simulink model "EV6_LUT_FourWheel_EV6Battery77p4kWh_PowerCorrected"  (R2024a)
settings: Solver=ode4  StartTime=0  StopTime=60  FixedStep=0.001  RelTol=1e-3
PreLoadFcn:
  | VSS_BICYCLE=Simulink.Variant('Dual=0');
  | VSS_DUAL=Simulink.Variant('Dual=1');
  | Dual=1;
  | load('DriveCycle2.mat')
PostLoadFcn:
  | if any(exist('dsrtsu_mdlpostloadfcn', 'file') ~= 0), dsrtsu_mdlpostloadfcn('Execute', bdroot); end
InitFcn:
  | , if any(exist('rtifpga_mdlclblib', 'file') ~= 0), rtifpga_mdlclblib('Init', bdroot); end,
  | , if any(exist('dsmpb_private', 'file') ~= 0), dsmpb_private('dsmpb_mdlclblib', 'Init', bdroot); end,
  | load('DriveCycle2.mat')
model workspace (MAT data in the model file):
  DiffRatio = 10.65
  EV6_2023_BattBranchCapacity_Ah = 55.5236728838
  EV6_2023_BattEnergy_kWh = 77.4
  EV6_2023_BattNominalVoltage_V = 697
  EV6_2023_BattNumCellsParallel = 2
  EV6_2023_BattNumCellsSeries = 192
  EV6_2023_BattOpenVoltCapBpts = [0 0.1 0.2 0.3 0.4 0.5 0.6 0.7 0.8 0.9 1]
  EV6_2023_BattOpenVoltTbl = [2.96762142548 3.40364281191 3.47417488548 3.54470541822 3.61523441014 3.68576186124 3.75628777151 3.82681214095 3.94527005036 4.07101207308 4.2120755254]
  EV6_2023_BattPackCapacity_Ah = 111.047345768
  EV6_2023_BattResistSocBpts = [0 0.2 0.4 0.6 0.8 1]
  EV6_2023_BattResistTbl = [0.0163620057716 0.0118174152018 0.00807187352333 0.00375663957972 0.00266904525531 0.00103635901355 0.0019014404175 0.0172368903217 0.0121226074867 0.00758541551769 0.00474065349228 0.00337561163613 ... (42 elements, 7x6)]
  EV6_2023_BattResistTempBpts = [243.1 253.1 263.1 273.1 283.1 298.1 313.1]
  EV6_2023_InitialPackOCV_V = 726.471714233
  EV6_2023_InitialSOC = 0.638878863672
  EV6_BattCellCapacity_Ah = 60.3
  EV6_BattInitialSOC = 0.638878863672
  EV6_BattOCV_Cell_V = [2.96762142548 3.40364281191 3.47417488548 3.54470541822 3.61523441014 3.68576186124 3.75628777151 3.82681214095 3.94527005036 4.07101207308 4.2120755254]
  EV6_BattOCV_SOC = [0 0.1 0.2 0.3 0.4 0.5 0.6 0.7 0.8 0.9 1]
  EV6_BattPackCapacity_Ah = 120.6
  EV6_BattParallelCells = 2
  EV6_BattResistanceSOC = [0 0.2 0.4 0.6 0.8 1]
  EV6_BattResistanceTable_Ohm = [0.0163620057716 0.0118174152018 0.00807187352333 0.00375663957972 0.00266904525531 0.00103635901355 0.0019014404175 0.0172368903217 0.0121226074867 0.00758541551769 0.00474065349228 0.00337561163613 ... (42 elements, 7x6)]
  EV6_BattResistanceTemp_K = [243.1 253.1 263.1 273.1 283.1 298.1 313.1]
  EV6_BattSeriesCells = 192
  EV6_FinalDriveRatio = 10.65
  EV6_TargetPackResistance_Ohm = 0.132763804608
  Gas = 0.383333333333
undefined symbols (not defined in the file): accel_bp_mps2, AccelCmd, ActTqLF_Nm_, ActTqLR_Nm_, ActTqRF_Nm_, ActTqRR_Nm_, BattChargeLimitMaxPwr, BattChargeLimitSocBpts, BattChargeLimitTbl, BattDischargeLimitSocBpts, BattDischargeLimitTbl, BattDischargeMaxPwr, BrakeMaxPrs, BrakeMaxTrq, ChassisDistCg2FrontAxle, ChassisDistCg2RearAxle, ChassisVehMass, CltchCmd, CoastDown, DecelCmd, DiscIntNeverNeededParam, EnvGravCnst, EnvPrs, EnvTemp, EV6_RegenTorqueGain, EV6_TractionTorqueGain, front_share_regen_3d, front_share_traction_3d, FuelSpecificGrav, GearCmd, h, InitStates, lgSw, limitedMCT, MCT, MtrEffSpdBpts, MtrEffTbl, MtrEffTrqBpts, MtrPwrMax, MtrTrqMax, out_1, pMCT, RealSimPara, Ref_speed, Ref_time, regen_torque_bp_Nm, speed_bp_kph, SteeringCmd, SupvsryCtrlRegenBrkCutOffTbl, SupvsryCtrlRegenSpdBpts, TestScnrioCycleNum, traction_torque_bp_Nm, US06, VEH
libraries: VSIGenLib x65, simulink x54, etargetslib x38, dsmpblib x24, vehdynlibtire x12, autolibshared x11, vehdynlibsuspension x7, vehdynlibtirecommon x7, autolibpowerinfoutils x6, autolibutils x5, autolibsharedcoupling x4, autolibmappedmotor x4
(part 15 of 19)

== system EV6_LUT_FourWheel_EV6Battery77p4kWh_PowerCorrected/Vehicle Under Test1/Vehicle/Vehicle Dynamics/Vehicle 7DOF/Longitudinal Wheels 4DOF/Veh2Tire/Wheel to Body Transform ==
  VelVeh : Inport  Partition=on  PartitionDimension=2  PartitionWidth=1  PartitionOffset=0
  WhlAng : Inport  Port=2  Partition=on  PartitionDimension=2  PartitionWidth=1  PartitionOffset=0
  Demux1 : Demux  Outputs=3
  Divide1 : Product  Inputs=**  Multiplication=Matrix(*)
  For Each : ForEach  DisableCoverage=on
  Rotation Angles to Direction Cosine Matrix : sharedtransform/Rotation Angles to Direction Cosine Matrix  rotationOrder=ZYX  aMode=2
  Selector : Selector  InputPortWidth=3  IndexOptions=Index vector (dialog)  Indices=[3 2 1]  OutputSizes=1
  xdotWheel : Outport  ConcatenationDimension=1  VectorParamsAs1DForOutWhenUnconnected=off
  ydotWheel : Outport  Port=2  ConcatenationDimension=1  VectorParamsAs1DForOutWhenUnconnected=off
  zdotWheel : Outport  Port=3  ConcatenationDimension=1  VectorParamsAs1DForOutWhenUnconnected=off
  wires:
  Selector/1 -> Rotation Angles to Direction Cosine Matrix/1
  WhlAng/1 -> Selector/1
  VelVeh/1 -> Divide1/2
  Rotation Angles to Direction Cosine Matrix/1 -> Divide1/1
  Demux1/3 -> zdotWheel/1
  Demux1/2 -> ydotWheel/1
  Demux1/1 -> xdotWheel/1
  Divide1/1 -> Demux1/1

== system EV6_LUT_FourWheel_EV6Battery77p4kWh_PowerCorrected/Vehicle Under Test1/Vehicle/Vehicle Dynamics/Vehicle 7DOF/Longitudinal Wheels 4DOF/Velocity and Vertical Load/Bicycle ==
  VehFdbk : Inport
  Bicycle Fz : Subsystem
  Bicycle V : Subsystem
  VehVel : Outport  VectorParamsAs1DForOutWhenUnconnected=off
  Fz : Outport  Port=2  VectorParamsAs1DForOutWhenUnconnected=off
  wires:
  VehFdbk/1 -> Bicycle V/1(In1), Bicycle Fz/1(In1)
  Bicycle Fz/1(Out1) -> Fz/1
  Bicycle V/1(Out1) -> VehVel/1

== system EV6_LUT_FourWheel_EV6Battery77p4kWh_PowerCorrected/Vehicle Under Test1/Vehicle/Vehicle Dynamics/Vehicle 7DOF/Longitudinal Wheels 4DOF/Velocity and Vertical Load/Dual ==
  VehFdbk : Inport
  Dual Fz : Subsystem
  Dual V : Subsystem
  VehVel : Outport  VectorParamsAs1DForOutWhenUnconnected=off
  Fz : Outport  Port=2  VectorParamsAs1DForOutWhenUnconnected=off
  wires:
  Dual Fz/1(Out1) -> Fz/1
  VehFdbk/1 -> Dual V/1(In1), Dual Fz/1(In1)
  Dual V/1(Out1) -> VehVel/1

== system EV6_LUT_FourWheel_EV6Battery77p4kWh_PowerCorrected/Vehicle Under Test1/Vehicle/Vehicle Dynamics/Vehicle 7DOF/Vehicle Body 3DOF External Longitudinal Wheels/Bicycle/Wheel Positions ==
  Info : Inport
  Bus Selector : BusSelector  OutputSignals=InertFrm.FrntAxl.Disp.Y,InertFrm.RearAxl.Disp.Y
  Bus Selector1 : BusSelector  OutputSignals=InertFrm.FrntAxl.Disp.X,InertFrm.RearAxl.Disp.X
  Constant : Constant  Value=0
  Constant1 : Constant  Value=0
  Vector Concatenate1 : Concatenate  NumInputs=4
  Vector Concatenate2 : Concatenate  NumInputs=4
  XWheel : Outport  Unit=m  VectorParamsAs1DForOutWhenUnconnected=off
  YWheel : Outport  Port=2  Unit=m  VectorParamsAs1DForOutWhenUnconnected=off
  wires:
  Bus Selector1/1 -> Vector Concatenate2/1  "<X>"
  Bus Selector1/2 -> Vector Concatenate2/3  "<X>"
  Vector Concatenate2/1 -> XWheel/1
  Info/1 -> Bus Selector1/1, Bus Selector/1
  Constant/1 -> Vector Concatenate2/2, Vector Concatenate2/4
  Bus Selector/1 -> Vector Concatenate1/1  "<Y>"
  Bus Selector/2 -> Vector Concatenate1/3  "<Y>"
  Vector Concatenate1/1 -> YWheel/1
  Constant1/1 -> Vector Concatenate1/2, Vector Concatenate1/4

== system EV6_LUT_FourWheel_EV6Battery77p4kWh_PowerCorrected/Vehicle Under Test1/Vehicle/Vehicle Dynamics/Vehicle 7DOF/Vehicle Body 3DOF External Longitudinal Wheels/Dual/Wheel Positions ==
  Info : Inport
  Bus Selector : BusSelector  OutputSignals=InertFrm.FrntAxl.Lft.Disp.Y,InertFrm.FrntAxl.Rght.Disp.Y,InertFrm.RearAxl.Lft.Disp.Y,InertFrm.RearAxl.Rght.Disp.Y
  Bus Selector1 : BusSelector  OutputSignals=InertFrm.FrntAxl.Lft.Disp.X,InertFrm.FrntAxl.Rght.Disp.X,InertFrm.RearAxl.Lft.Disp.X,InertFrm.RearAxl.Rght.Disp.X
  Vector Concatenate1 : Concatenate  NumInputs=4
  Vector Concatenate2 : Concatenate  NumInputs=4
  XWheel : Outport  Unit=m  VectorParamsAs1DForOutWhenUnconnected=off
  YWheel : Outport  Port=2  Unit=m  VectorParamsAs1DForOutWhenUnconnected=off
  wires:
  Vector Concatenate2/1 -> XWheel/1
  Bus Selector1/1 -> Vector Concatenate2/1  "<X>"
  Info/1 -> Bus Selector1/1, Bus Selector/1
  Vector Concatenate1/1 -> YWheel/1
  Bus Selector/2 -> Vector Concatenate1/2  "<Y>"
  Bus Selector/3 -> Vector Concatenate1/3  "<Y>"
  Bus Selector1/2 -> Vector Concatenate2/2  "<X>"
  Bus Selector/4 -> Vector Concatenate1/4  "<Y>"
  Bus Selector1/3 -> Vector Concatenate2/3  "<X>"
  Bus Selector/1 -> Vector Concatenate1/1  "<Y>"
  Bus Selector1/4 -> Vector Concatenate2/4  "<X>"

== system EV6_LUT_FourWheel_EV6Battery77p4kWh_PowerCorrected/Vehicle Under Test1/Vehicle/Battery/Battery/Lithium Ion Battery Pack1/Datasheet Battery Internal/Datasheet Battery/Charge Model ==
  LdAmp : Inport
  CapInit : Inport  Port=2
  Constant1 : Constant  Value=BattChargeMax
  Gain1 : Gain  Gain=-1/(Np*3600)
  Integrator Limited : Integrator  InitialConditionSource=external  InitialCondition=BattCapInit  LimitOutput=on  UpperSaturationLimit=BattChargeMax  LowerSaturationLimit=0
  Switch : Switch  Criteria=u2 > Threshold  Threshold=BattChargeMax  SaturateOnIntegerOverflow=off  InputSameDT=off
  LdAmpHr : Outport  VectorParamsAs1DForOutWhenUnconnected=off
  wires:
  Gain1/1 -> Integrator Limited/1
  Integrator Limited/1 -> LdAmpHr/1
  LdAmp/1 -> Gain1/1
  CapInit/1 -> Switch/3, Switch/2
  Constant1/1 -> Switch/1
  Switch/1 -> Integrator Limited/2

== system EV6_LUT_FourWheel_EV6Battery77p4kWh_PowerCorrected/Vehicle Under Test1/Vehicle/Battery/Battery/Lithium Ion Battery Pack1/Datasheet Battery Internal/Datasheet Battery/State of Charge Capacity ==
  LdAmpHr : Inport
  Constant1 : Constant  Value=BattChargeMax
  Divide : Product  Inputs=*/
  CapSOC : Outport  VectorParamsAs1DForOutWhenUnconnected=off
  wires:
  Constant1/1 -> Divide/2
  LdAmpHr/1 -> Divide/1
  Divide/1 -> CapSOC/1

== system EV6_LUT_FourWheel_EV6Battery77p4kWh_PowerCorrected/Vehicle Under Test1/Vehicle/Battery/Battery/Lithium Ion Battery Pack1/Datasheet Battery Internal/Datasheet Battery/Voltage and Power Calculation ==
  CapSOC : Inport
  LdAmp : Inport  Port=2
  BattTemp : Inport  Port=3
  Em : Lookup_n-D  NumberOfTableDimensions=1  LookupTableObject=''  BreakpointsForDimension1=CapLUTBp  BreakpointsForDimension2=CapSOCBp  Table=Em  ExtrapMethod=Clip  UseLastTableValue=on  InternalRulePriority=Speed  RndMeth=Simplest
  Gain1 : Gain  Gain=Ns
  Gain2 : Gain  Gain=1/Np
  Gain3 : Gain  Gain=Ns
  Gain4 : Gain  Gain=Np
  Product : Product
  Product1 : Product
  R : Lookup_n-D  LookupTableObject=''  BreakpointsForDimension1=BattTempBp  BreakpointsForDimension2=CapSOCBp  Table=RInt  ExtrapMethod=Clip  UseLastTableValue=on  InternalRulePriority=Speed  RndMeth=Simplest
      settings: InputPortMap=u0,u1
  Subtract : Sum  Inputs=+-
  OutVolt : Outport  VectorParamsAs1DForOutWhenUnconnected=off
  BattPwrLoss : Outport  Port=2  VectorParamsAs1DForOutWhenUnconnected=off
  wires:
  Gain1/1 -> OutVolt/1
  Em/1 -> Subtract/1
  R/1 -> Product/1
  Product/1 -> Product1/1, Subtract/2
  BattTemp/1 -> R/1
  Subtract/1 -> Gain1/1
  LdAmp/1 -> Gain2/1
  CapSOC/1 -> Em/1, R/2
  Gain2/1 -> Product1/2, Product/2
  Product1/1 -> Gain3/1
  Gain3/1 -> Gain4/1
  Gain4/1 -> BattPwrLoss/1

== system EV6_LUT_FourWheel_EV6Battery77p4kWh_PowerCorrected/Vehicle Under Test1/Vehicle/Driver and Drive Cycle/Driver and PI with FF Control/Speed controller set/Predictive/Longitudinal Driver1/Longitudinal Driver ==
  Vref : Inport
  Vfdbk : Inport  Port=2
  Grade : Inport  Port=3
  Longitudinal Driver Model : autolibshared/Longitudinal Driver  extAccelOvr=off  extDecelOvr=off  extAccelHld=off  extDecelHld=off  extAccelZero=off  extDecelZero=off  cntrlType=Predictive  shftType=Reverse, Neutral, Drive  velUnits=m/s  gearOut=off  Kp=1  Ki=1  Kff=0  Kg=0  VehVelVec=[0 100]  KffVec=[.1 .1]  KpVec=[10 10]  KiVec=[5 5]  KgVec=[0 0]  m=1500  Kpt=Kpt  tau=tau  L=L  aR=160  bR=1  cR=0.36  g=9.81  vnom=1  Kaw=0  tauerr=0  tauPt=2  GearInit=0  tShift=.1  pdlVec=[0.1 0.4 0.5 0.9]  upShftTbl=[-1 12.9375 26.4375 39.9375 51.18749999999999 62.4375 72.84375 83.25;-1 16.3125 29.8125 43.3125 54.5624 65.8125 76.78125 87.75;-1 19.6875 33.1875 46.68749999999999 57.9375 69.1875 80.71875 92.25;-1 33 52.5 77.25 100.5 138.75 161.875 185]  dwnShftTbl=[1 9.5625 23.0625 36.5625 47.8125 59.0625 68.90625 78.75;1 12.9375 26.4375 39.9375 51.18749999999999 62.4375 72.84375 83.25;1 16.3125 29.8125 43.3125 54.562499 65.8125 76.78125 87.75;1 19.6875 33.1875 46.68749999999999 57.9375 69.1875 80.71875 92.25]  tClutch=.5  tRev=.5  tPark=120  aMode=1  UpGearVec="[0  1  2  3  4  5  6  7]"  DownGearVec="[1  2  3  4  5  6  7  8]"
  OpCmds : Outport  VectorParamsAs1DForOutWhenUnconnected=off
  Acc : Outport  Port=2  VectorParamsAs1DForOutWhenUnconnected=off
  Dec : Outport  Port=3  VectorParamsAs1DForOutWhenUnconnected=off
  wires:
  Longitudinal Driver Model/1 -> OpCmds/1  "Info"
  Grade/1 -> Longitudinal Driver Model/3
  Longitudinal Driver Model/3 -> Dec/1  "Dec"
  Longitudinal Driver Model/2 -> Acc/1  "Acc"
  Vref/1 -> Longitudinal Driver Model/1  "xdotref"
  Vfdbk/1 -> Longitudinal Driver Model/2

== system EV6_LUT_FourWheel_EV6Battery77p4kWh_PowerCorrected/Vehicle Under Test1/Vehicle/Driver and Drive Cycle/Driver and PI with FF Control/Speed controller set/Predictive/Longitudinal Driver1/Open Loop ==
  note: This subsystem is provided to disable the driver subsystem and expose the driver interface.
      |
      | The interface can:
      | - be connected with dashboard UI blocks or 3rd party hardware
      | - provide application specific pre-programmed event or time based signals
      | - be driven by recorded operator signals for tuning, troubleshooting and model validation
  Bus Creator2 : BusCreator  Inputs=8
  Constant{1..4} (4 alike) : Constant  Value=0
  Ground{,1..3} (4 alike) : Ground
  OpCmds : Outport  VectorParamsAs1DForOutWhenUnconnected=off
  wires:
  Constant4/1 -> Bus Creator2/4  "Clutch"
  Ground/1 -> Bus Creator2/5  "Err"
  Constant2/1 -> Bus Creator2/2  "Decel"
  Constant3/1 -> Bus Creator2/3  "Gear"
  Constant1/1 -> Bus Creator2/1  "Accel"
  Ground2/1 -> Bus Creator2/7  "ErrMax"
  Bus Creator2/1 -> OpCmds/1  "Info"
  Ground1/1 -> Bus Creator2/6  "ErrSqrSum"
  Ground3/1 -> Bus Creator2/8  "ErrMin"

== system EV6_LUT_FourWheel_EV6Battery77p4kWh_PowerCorrected/Vehicle Under Test1/Vehicle/Driver and Drive Cycle/Driver and PI with FF Control/Speed controller set/Speed tracking controller/In-house CAVE/Vehicle Speed Controller ==
  note: ToDo: Maybe do something clever with FF and Brake, or maybe not.
      | Bleed FF based on refspd derivative
  RefSpd : Inport
  VehicleSpeed : Inport  Port=2
  Add : Sum  Inputs=+-
  Compare To Constant1 : simulink/Logic and Bit Operations/Compare To Constant  relop=<=  const=0.1  OutDataTypeStr=boolean  ZeroCross=off
  Compare To Constant3 : simulink/Logic and Bit Operations/Compare To Constant  relop=<=  const=0  OutDataTypeStr=boolean  ZeroCross=off
  Constant : Constant  Value=0
  Detect Fall Negative : simulink/Logic and Bit Operations/Detect Fall Negative  vinit=0  OutDataTypeStr=boolean
  Detect Rise Positive : simulink/Logic and Bit Operations/Detect Rise Positive  vinit=0  OutDataTypeStr=boolean
  Feedforward : Lookup_n-D  NumberOfTableDimensions=1  BreakpointsForDimension1="[0 10    20    30    40    50    60    70    80    90   100   110   120   130   140   150   160]"  Table="[0\t3.5\t12.5\t16\t20\t21\t22\t24.5\t26\t29.5\t32\t33\t34\t36\t37\t38\t39]"  ExtrapMethod=Clip  InternalRulePriority=Speed  RndMeth=Simplest
  Feedforward1 : Lookup_n-D  NumberOfTableDimensions=1  BreakpointsForDimension1="[0 10    20    30    40    50    60    70    80    90   100   110   120   130   140   150   160]"  Table="[0 2.6021    4.7790    6.8575    8.1555    9.4176   10.7914   12.3245   14.1570   15.9699   17.4605   19.0355   21.3079   22.8407   25.3373   26.9453   28.6975]"  ExtrapMethod=Clip  InternalRulePriority=Speed  RndMeth=Simplest
  FeedforwardGain : Gain
  Gain : Gain  Gain=-1
  Ground1 : Ground
  Ki : Gain
  Kp : Gain  Gain=10
  Limits [-50,50] : Integrator  ExternalReset=either  LimitOutput=on  UpperSaturationLimit=50  LowerSaturationLimit=-50
  Logical Operator : Logic  Operator=OR  Inputs=3  AllPortsSameDT=off  OutDataTypeStr=boolean
  Lowpass Filter : TransferFcn  Denominator=[.02 1]
  Memory : Memory
  Memory1 : Memory
  Min threshold for Brake switch : Constant  Value=0
  Product1 : Product  RndMeth=Zero
  Proportional Gain Scheduling : Lookup_n-D  NumberOfTableDimensions=1  BreakpointsForDimension1=[ 0 30 70]  IndexSearchMethod=Linear search  BeginIndexSearchUsingPreviousIndexResult=on  Table=[1 1 1]  ExtrapMethod=Clip  UseLastTableValue=on  RndMeth=Simplest
  Relational Operator : RelationalOperator  Operator=>  OutDataTypeStr=boolean  InputSameDT=off
  Sum : Sum  Inputs=|+-
  Sum1 : Sum  Inputs=+++
  Switch{1..4} (4 alike) : Switch  Criteria=u2 > Threshold  SaturateOnIntegerOverflow=off  InputSameDT=off
  standstill brake [0,100] : Constant  Value=50
  AcceleratorPedalPos : Outport  VectorParamsAs1DForOutWhenUnconnected=off
  BrakePedalPos : Outport  Port=2  VectorParamsAs1DForOutWhenUnconnected=off
  BrakeSwitch : Outport  Port=3  VectorParamsAs1DForOutWhenUnconnected=off
  wires:
  FeedforwardGain/1 -> Sum1/3  "Driver_FdfwdTerm_pct"
  Feedforward1/1 -> FeedforwardGain/1
  Product1/1 -> Sum1/2  "Driver_PropTerm_pct"
  Proportional Gain Scheduling/1 -> Product1/2
  Switch4/1 -> BrakePedalPos/1  "BrakePedalPos_pct"
  standstill brake [0,100]/1 -> Switch4/1
  Constant/1 -> Switch3/1
  Switch3/1 -> AcceleratorPedalPos/1  "AcceleratorPedalPos_pct"
  Compare To Constant1/1 -> Switch4/2, Switch3/2
  Memory1/1 -> Add/1
  Memory/1 -> Add/2
  Add/1 -> Detect Rise Positive/1, Detect Fall Negative/1
  Detect Fall Negative/1 -> Logical Operator/3
  Detect Rise Positive/1 -> Logical Operator/2
  Compare To Constant3/1 -> Logical Operator/1
  Logical Operator/1 -> Limits [-50,50]/2
  Gain/1 -> Switch2/2, Switch2/1
  Ground1/1 -> Switch1/3, Switch2/3
  Ki/1 -> Limits [-50,50]/1
  Sum1/1 -> Switch1/2, Switch1/1, Gain/1  "Driver_TotCmdPreLim_pct"
  Relational Operator/1 -> BrakeSwitch/1  "BrakeSwitch"
  Lowpass Filter/1 -> Sum/2  "VS_Flt"
  Switch2/1 -> Memory/1, Relational Operator/1, Switch4/3  "BrakePedalPosPre_pct"
  VehicleSpeed/1 -> Lowpass Filter/1, Proportional Gain Scheduling/1
  Limits [-50,50]/1 -> Sum1/1  "Driver_IntTerm_pct"
  Sum/1 -> Ki/1, Kp/1  "SpdErr"
  RefSpd/1 -> Sum/1, Compare To Constant3/1, Compare To Constant1/1, Feedforward1/1  "RefSpd"
  Switch1/1 -> Memory1/1, Switch3/3  "AcceleratorPedalPosPre_pct"
  Min threshold for Brake switch/1 -> Relational Operator/2
  Kp/1 -> Product1/1

== system EV6_LUT_FourWheel_EV6Battery77p4kWh_PowerCorrected/Vehicle Under Test1/Vehicle/Vehicle Dynamics/Vehicle 14DOF/Wheels and Tires/VDBS/Tire2Veh/Routiong ==
  <Mz> : Inport
  <Mx> : Inport  Port=2
  <My> : Inport  Port=3
  <Re> : Inport  Port=4
  <z> : Inport  Port=5
  <zdot> : Inport  Port=6
  <Kappa> : Inport  Port=7
  <Alpha> : Inport  Port=8
  Omega : Inport  Port=9
  Fx : Inport  Port=10
  Fy : Inport  Port=11
  Fz : Inport  Port=12
  Bus Creator : BusCreator  Inputs=12
  Reshape : Reshape  OutputDimensionality=Row vector (2-D)
  Reshape1 : Reshape  OutputDimensionality=Row vector (2-D)
  Unary Minus1 : UnaryMinus
  Unary Minus2 : UnaryMinus
  Out1 : Outport  VectorParamsAs1DForOutWhenUnconnected=off
  Out2 : Outport  Port=2  VectorParamsAs1DForOutWhenUnconnected=off
  Out3 : Outport  Port=3  VectorParamsAs1DForOutWhenUnconnected=off
  wires:
  <Alpha>/1 -> Bus Creator/12
  <My>/1 -> Bus Creator/6
  <Mx>/1 -> Bus Creator/5
  Reshape/1 -> Out2/1
  <Kappa>/1 -> Bus Creator/11
  Reshape1/1 -> Out3/1
  Fx/1 -> Bus Creator/2
  Omega/1 -> Bus Creator/1  "Omega"
  Fy/1 -> Bus Creator/3
  Bus Creator/1 -> Out1/1
  <z>/1 -> Unary Minus1/1
  Unary Minus2/1 -> Bus Creator/10, Reshape1/1  "zdot"
  <Mz>/1 -> Bus Creator/7
  <zdot>/1 -> Unary Minus2/1
  Fz/1 -> Bus Creator/4
  Unary Minus1/1 -> Bus Creator/9, Reshape/1  "z"
  <Re>/1 -> Bus Creator/8

== system EV6_LUT_FourWheel_EV6Battery77p4kWh_PowerCorrected/Vehicle Under Test1/Vehicle/Vehicle Dynamics/Vehicle 14DOF/Wheels and Tires/VDBS/Tire2Veh/Wheel Angles ==
  Front : Inport
  Camber : Inport  Port=2
  Add1 : Sum
  Add2 : Sum
  Constant1 : Constant  Value=pi
  Constant2 : Constant  Value=[pi;0;pi;0].*0+[0;pi;0;pi].*.0
  Constant3 : Constant  Value=ones(1,4).*0
  Reshape : Reshape  OutputDimensionality=Row vector (2-D)
  Reshape1 : Reshape  OutputDimensionality=Row vector (2-D)
  Reshape2 : Reshape  OutputDimensionality=Row vector (2-D)
  Vector Concatenate3 : Concatenate  NumInputs=3  Mode=Multidimensional array
  Vehicle : Outport  VectorParamsAs1DForOutWhenUnconnected=off
  wires:
  Constant1/1 -> Add2/2
  Add2/1 -> Reshape1/1
  Camber/1 -> Add2/1
  Add1/1 -> Reshape/1
  Constant3/1 -> Reshape2/1
  Reshape1/1 -> Vector Concatenate3/1
  Front/1 -> Add1/1
  Constant2/1 -> Add1/2
  Vector Concatenate3/1 -> Vehicle/1
  Reshape2/1 -> Vector Concatenate3/2
  Reshape/1 -> Vector Concatenate3/3

== system EV6_LUT_FourWheel_EV6Battery77p4kWh_PowerCorrected/Vehicle Under Test1/Vehicle/Vehicle Dynamics/Vehicle 14DOF/Wheels and Tires/VDBS/Tire2Veh/Wheel to Body Transform ==
  Forces : Inport  Partition=on  PartitionDimension=2  PartitionWidth=1  PartitionOffset=0
  WheelAngles : Inport  Port=2  Partition=on  PartitionDimension=2  PartitionWidth=1  PartitionOffset=0
  Demux1 : Demux  Outputs=3
  Divide1 : Product  Inputs=**  Multiplication=Matrix(*)
  For Each : ForEach  DisableCoverage=on
  Rotation Angles to Direction Cosine Matrix Retro: ZYX : Subsystem
  Selector : Selector  InputPortWidth=3  IndexOptions=Index vector (dialog)  Indices=[3 2 1]  OutputSizes=1
  Fx : Outport  ConcatenationDimension=1  VectorParamsAs1DForOutWhenUnconnected=off
  Fy : Outport  Port=2  ConcatenationDimension=1  VectorParamsAs1DForOutWhenUnconnected=off
  Fz : Outport  Port=3  ConcatenationDimension=1  VectorParamsAs1DForOutWhenUnconnected=off
  wires:
  Selector/1 -> Rotation Angles to Direction Cosine Matrix Retro: ZYX/1(In1)
  WheelAngles/1 -> Selector/1
  Forces/1 -> Divide1/2
  Rotation Angles to Direction Cosine Matrix Retro: ZYX/1(Out1) -> Divide1/1
  Demux1/3 -> Fz/1
  Demux1/2 -> Fy/1
  Demux1/1 -> Fx/1
  Divide1/1 -> Demux1/1
